simulink model "gtm_design"  (R2021b)
settings: Solver=VariableStepAuto  StartTime=0.0  StopTime=10.0  MinStep=0.00999  RelTol=1e-3
StopFcn:
  | MWSout=grabmws(bdroot);
  | MWSout.lastrun=datestr(now);
values from neighbouring files (symbols this model uses):
  knots2fps = 1.68781    [setup.m]
  s = tf('s')    [setup.m]
undefined symbols (not defined in the file or in its folder): Aero, aftfuel, aftfuel_pos, AILL, AILLC, AILR, AILRC, alpha_deg, alt0, altitude_ft, Ax_g, Ay_g, Az_g, b, beta_deg, bias, BRAKEC, Cbar, cg_pos0, cg_shift_gear, ControlMode, DamageCase, DamageModels, DamageOnsetTime, deltc, Earth, ELLIB, ELLIBC, ELLOB, ELLOBC, ELRIB, ELRIBC, ELROB, ELROBC, engl_ang, engl_pos, engr_ang, engr_pos, etas0, etas1, etasc_feedthrough, FLAPLC, FLAPLIB, FLAPLOB, FLAPRC, FLAPRIB, FLAPROB, FlightMode, FuelUsed_Init, fwdfuel, fwdfuel_pos, GEAR, GEARC, Inertia0, Inertia_shift_gear, Ixx_model, Iyy_model, Izz_model, KTAS, LandingGear ... (+66)
libraries: simulink_extras x98, LPVBlockLibrary x54, simulink_need_slupdate x30, aerolibconvert2 x27, simulink x7, aerolibtransform2 x6, uavalgslib x4, UserContent_lib x2, robotcorelib x1, uavutilslib x1
(part 9 of 9)

== system gtm_design/Control/Controller/Control Algorithm/LPV Autopilot/Longitudinal Controller/Scheduling Parameter ==
  feedback : Inport
  Add : Sum
  Bus Selector1 : BusSelector  OutputSignals=AirData.KTAS,MIDG.NAV_altitude_m,SurfacePos.FLAPLOB,SurfacePos.FLAPROB  OutputAsBus=on
  Bus to Vector : BusToVector
  Demux : Demux
  Gain : Gain  Gain=0.5
  Length Conversion : aerolibconvert2/Length Conversion  IU=m  OU=ft
  MATLAB Function : MATLAB Function  TreatAsAtomicUnit=on
  Mux : Mux  Inputs=3
  rho : Outport
  wires:
  feedback/1 -> Bus Selector1/1
  Bus Selector1/1 -> Bus to Vector/1
  Demux/3 -> Add/1
  Demux/1 -> MATLAB Function/1(tas)
  Demux/4 -> Add/2
  MATLAB Function/1(sas) -> Mux/1  "sas"
  Add/1 -> Gain/1
  Gain/1 -> Mux/3  "mor"
  Demux/2 -> Length Conversion/1  "alt"
  Bus to Vector/1 -> Demux/1
  Mux/1 -> rho/1
  Length Conversion/1 -> MATLAB Function/2(h), Mux/2

== system gtm_design/Control/Controller/Control Algorithm/LPV Autopilot/Longitudinal Controller/Trim Command ==
  rho : Inport
  Constant4 : Constant
  Constant5 : Constant
  LPVBlock1 : LPVBlockLibrary/LPVBlock  sys=sch_param.sch_alt_trim  plist={'rho1_sas_param';'rho2_alt_param';'rho3_mor_param'}  x0=0
      settings: SourceProductName=LPVTools Blocks
  LPVBlock2 : LPVBlockLibrary/LPVBlock  sys=sch_param.sch_tas_trim  plist={'rho1_sas_param';'rho2_alt_param';'rho3_mor_param'}  x0=0
      settings: SourceProductName=LPVTools Blocks
  Mux : Mux  Inputs=2
  knotstofps : Gain  Gain=knots2fps
  r_eq : Outport
  wires:
  Mux/1 -> r_eq/1
  Constant5/1 -> LPVBlock2/1
  LPVBlock2/1 -> knotstofps/1  "tas_trim_knot"
  LPVBlock1/1 -> Mux/2  "alt_trim_ft"
  Constant4/1 -> LPVBlock1/1
  rho/1 -> LPVBlock2/2, LPVBlock1/2
  knotstofps/1 -> Mux/1  "tas_trim_fps"

== system gtm_design/Control/Controller/Control Algorithm/LPV Autopilot/Longitudinal Controller/Trim Input ==
  rho : Inport
  Constant1 : Constant
  Constant3 : Constant
  Mux : Mux  Inputs=2
  dele_trim : LPVBlockLibrary/LPVBlock  sys=sch_param.sch_elevator_trim  plist={'rho1_sas_param';'rho2_alt_param';'rho3_mor_param'}  x0=0
      settings: SourceProductName=LPVTools Blocks
  delt_trim : LPVBlockLibrary/LPVBlock  sys=sch_param.sch_throttle_trim  plist={'rho1_sas_param';'rho2_alt_param';'rho3_mor_param'}  x0=0
      settings: SourceProductName=LPVTools Blocks
  u_eq : Outport
  wires:
  Constant3/1 -> dele_trim/1
  dele_trim/1 -> Mux/2  "dele_trim_deg"
  rho/1 -> dele_trim/2, delt_trim/2
  delt_trim/1 -> Mux/1  "delt_trim_percent"
  Constant1/1 -> delt_trim/1
  Mux/1 -> u_eq/1

== system gtm_design/Control/Controller/Control Algorithm/LPV Autopilot/Longitudinal Controller/Trim State ==
  rho : Inport
  Constant{2..6} (5 alike) : Constant
  Degrees to Radians : simulink_extras/Transformations/Degrees to Radians
  Degrees to Radians1 : simulink_extras/Transformations/Degrees to Radians
  Degrees to Radians2 : simulink_extras/Transformations/Degrees to Radians
  LPVBlock : LPVBlockLibrary/LPVBlock  sys=sch_param.sch_alp_trim  plist={'rho1_sas_param';'rho2_alt_param';'rho3_mor_param'}  x0=0
      settings: SourceProductName=LPVTools Blocks
  LPVBlock1 : LPVBlockLibrary/LPVBlock  sys=sch_param.sch_alt_trim  plist={'rho1_sas_param';'rho2_alt_param';'rho3_mor_param'}  x0=0
      settings: SourceProductName=LPVTools Blocks
  LPVBlock2 : LPVBlockLibrary/LPVBlock  sys=sch_param.sch_tas_trim  plist={'rho1_sas_param';'rho2_alt_param';'rho3_mor_param'}  x0=0
      settings: SourceProductName=LPVTools Blocks
  LPVBlock3 : LPVBlockLibrary/LPVBlock  sys=sch_param.sch_qdeg_trim  plist={'rho1_sas_param';'rho2_alt_param';'rho3_mor_param'}  x0=0
      settings: SourceProductName=LPVTools Blocks
  Mux : Mux  Inputs=5
  knotstofps : Gain  Gain=knots2fps
  sch_pitch_trim : LPVBlockLibrary/LPVBlock  sys=sch_param.sch_pitch_trim  plist={'rho1_sas_param';'rho2_alt_param';'rho3_mor_param'}  x0=0
      settings: SourceProductName=LPVTools Blocks
  x_eq : Outport
  wires:
  Constant5/1 -> LPVBlock2/1
  LPVBlock1/1 -> Mux/5  "alt_trim_deg"
  Constant4/1 -> LPVBlock1/1
  Mux/1 -> x_eq/1
  Degrees to Radians1/1 -> Mux/4  "theta_trim_rad"
  Constant3/1 -> sch_pitch_trim/1
  sch_pitch_trim/1 -> Degrees to Radians1/1  "theta_trim_deg"
  LPVBlock/1 -> Degrees to Radians/1  "alp_trim_deg"
  Constant2/1 -> LPVBlock/1
  LPVBlock2/1 -> knotstofps/1  "tas_trim_knot"
  Degrees to Radians/1 -> Mux/2  "alp_trim_rad"
  knotstofps/1 -> Mux/1  "tas_trim_fps"
  Constant6/1 -> LPVBlock3/1
  rho/1 -> LPVBlock/2, LPVBlock3/2, sch_pitch_trim/2, LPVBlock1/2, LPVBlock2/2
  LPVBlock3/1 -> Degrees to Radians2/1  "q_trim_deg"
  Degrees to Radians2/1 -> Mux/3  "q_trim_rad"

== system gtm_design/Control/Controller/Control Algorithm/LPV CAS/Lateral-Directional Controller/Full State ==
  feedback : Inport
  Bus Selector : BusSelector  OutputSignals=AirData.beta_deg,MAG3.p_deg,MAG3.r_deg
  Degrees to Radians : simulink_extras/Transformations/Degrees to Radians
  Degrees to Radians1 : simulink_extras/Transformations/Degrees to Radians
  Degrees to Radians2 : simulink_extras/Transformations/Degrees to Radians
  Mux : Mux  Inputs=3
  x : Outport
  wires:
  feedback/1 -> Bus Selector/1
  Bus Selector/1 -> Degrees to Radians2/1  "<beta_deg>"
  Bus Selector/2 -> Degrees to Radians/1  "<p_deg>"
  Bus Selector/3 -> Degrees to Radians1/1  "<r_deg>"
  Degrees to Radians1/1 -> Mux/3  "r_rad"
  Degrees to Radians/1 -> Mux/2  "p_rad"
  Degrees to Radians2/1 -> Mux/1  "bet_rad"
  Mux/1 -> x/1

== system gtm_design/Control/Controller/Control Algorithm/LPV CAS/Lateral-Directional Controller/Scheduling Parameter ==
  feedback : Inport
  Add : Sum
  Bus Selector1 : BusSelector  OutputSignals=AirData.KTAS,MIDG.NAV_altitude_m,SurfacePos.FLAPLOB,SurfacePos.FLAPROB  OutputAsBus=on
  Bus to Vector : BusToVector
  Demux : Demux
  Gain : Gain  Gain=0.5
  Length Conversion : aerolibconvert2/Length Conversion  IU=m  OU=ft
  MATLAB Function : MATLAB Function  TreatAsAtomicUnit=on
  Mux : Mux  Inputs=3
  rho : Outport
  wires:
  feedback/1 -> Bus Selector1/1
  Bus Selector1/1 -> Bus to Vector/1
  Demux/3 -> Add/1
  Demux/1 -> MATLAB Function/1(tas)
  Demux/4 -> Add/2
  MATLAB Function/1(sas) -> Mux/1  "sas"
  Add/1 -> Gain/1
  Gain/1 -> Mux/3  "mor"
  Demux/2 -> Length Conversion/1  "alt"
  Bus to Vector/1 -> Demux/1
  Mux/1 -> rho/1
  Length Conversion/1 -> MATLAB Function/2(h), Mux/2

== system gtm_design/Control/Controller/Control Algorithm/LPV CAS/Lateral-Directional Controller/Trim Command ==
  rho : Inport
  Constant : Constant  Value=0
  Constant1 : Constant  Value=0
  Degrees to Radians : simulink_extras/Transformations/Degrees to Radians
  Degrees to Radians1 : simulink_extras/Transformations/Degrees to Radians
  Mux : Mux  Inputs=2
  Terminator : Terminator
  r_eq : Outport
  wires:
  Degrees to Radians1/1 -> Mux/2
  Degrees to Radians/1 -> Mux/1
  Constant1/1 -> Degrees to Radians1/1  "p_trim"
  Constant/1 -> Degrees to Radians/1  "bet_trim"
  rho/1 -> Terminator/1
  Mux/1 -> r_eq/1

== system gtm_design/Control/Controller/Control Algorithm/LPV CAS/Lateral-Directional Controller/Trim Input ==
  rho : Inport
  Constant1 : Constant  Value=0
  Constant2 : Constant
  Constant3 : Constant
  LPVBlock : LPVBlockLibrary/LPVBlock  sys=sch_param.sch_aileron_trim  plist={'rho1_sas_param';'rho2_alt_param';'rho3_mor_param'}  x0=0
      settings: SourceProductName=LPVTools Blocks
  LPVBlock1 : LPVBlockLibrary/LPVBlock  sys=sch_param.sch_rudder_trim  plist={'rho1_sas_param';'rho2_alt_param';'rho3_mor_param'}  x0=0
      settings: SourceProductName=LPVTools Blocks
  Mux : Mux  Inputs=3
  x_eq : Outport
  wires:
  Constant3/1 -> LPVBlock1/1
  Mux/1 -> x_eq/1
  rho/1 -> LPVBlock/2, LPVBlock1/2
  Constant2/1 -> LPVBlock/1
  LPVBlock1/1 -> Mux/2  "delr_trim_deg"
  Constant1/1 -> Mux/3  "etaa_trim_deg"
  LPVBlock/1 -> Mux/1  "dela_trim_deg"

== system gtm_design/Control/Controller/Control Algorithm/LPV CAS/Lateral-Directional Controller/Trim State ==
  rho : Inport
  Constant1 : Constant
  Constant2 : Constant
  Constant3 : Constant
  Degrees to Radians : simulink_extras/Transformations/Degrees to Radians
  Degrees to Radians1 : simulink_extras/Transformations/Degrees to Radians
  Degrees to Radians2 : simulink_extras/Transformations/Degrees to Radians
  LPVBlock : LPVBlockLibrary/LPVBlock  sys=sch_param.sch_beta_trim  plist={'rho1_sas_param';'rho2_alt_param';'rho3_mor_param'}  x0=0
      settings: SourceProductName=LPVTools Blocks
  LPVBlock1 : LPVBlockLibrary/LPVBlock  sys=sch_param.sch_pdeg_trim  plist={'rho1_sas_param';'rho2_alt_param';'rho3_mor_param'}  x0=0
      settings: SourceProductName=LPVTools Blocks
  LPVBlock2 : LPVBlockLibrary/LPVBlock  sys=sch_param.sch_rdeg_trim  plist={'rho1_sas_param';'rho2_alt_param';'rho3_mor_param'}  x0=0
      settings: SourceProductName=LPVTools Blocks
  Mux : Mux  Inputs=3
  x_eq : Outport
  wires:
  Degrees to Radians/1 -> Mux/1  "beta_trim_rad"
  Constant2/1 -> LPVBlock/1
  LPVBlock/1 -> Degrees to Radians/1  "beta_trim_deg"
  LPVBlock1/1 -> Degrees to Radians1/1  "p_trim_deg"
  rho/1 -> LPVBlock2/2, LPVBlock1/2, LPVBlock/2
  Mux/1 -> x_eq/1
  Degrees to Radians1/1 -> Mux/2  "p_trim_rad"
  Constant3/1 -> LPVBlock1/1
  Constant1/1 -> LPVBlock2/1
  LPVBlock2/1 -> Degrees to Radians2/1  "r_trim_deg"
  Degrees to Radians2/1 -> Mux/3  "r_trim_rad"

== system gtm_design/Control/Controller/Control Algorithm/LPV CAS/Longitudinal Controller/Full State ==
  feedback : Inport
  Bus Selector : BusSelector  OutputSignals=AirData.alpha_deg,MAG3.q_deg,MAG3.Az_g
  Degrees to Radians : simulink_extras/Transformations/Degrees to Radians
  Degrees to Radians1 : simulink_extras/Transformations/Degrees to Radians
  Mux : Mux  Inputs=3
  knotstofps : Gain  Gain=32.174
  y : Outport
  wires:
  knotstofps/1 -> Mux/3  "Az_ft/s^2"
  Degrees to Radians1/1 -> Mux/2  "q_rad"
  Degrees to Radians/1 -> Mux/1  "alp_rad"
  Mux/1 -> y/1
  Bus Selector/3 -> knotstofps/1  "<Az_g>"
  Bus Selector/2 -> Degrees to Radians1/1  "<q_deg>"
  Bus Selector/1 -> Degrees to Radians/1  "<alpha_deg>"
  feedback/1 -> Bus Selector/1

== system gtm_design/Control/Controller/Control Algorithm/LPV CAS/Longitudinal Controller/Scheduling Parameter ==
  feedback : Inport
  Add : Sum
  Bus Selector1 : BusSelector  OutputSignals=AirData.KTAS,MIDG.NAV_altitude_m,SurfacePos.FLAPLOB,SurfacePos.FLAPROB  OutputAsBus=on
  Bus to Vector : BusToVector
  Demux : Demux
  Gain : Gain  Gain=0.5
  Length Conversion : aerolibconvert2/Length Conversion  IU=m  OU=ft
  MATLAB Function : MATLAB Function  TreatAsAtomicUnit=on
  Mux : Mux  Inputs=3
  rho : Outport
  wires:
  Length Conversion/1 -> Mux/2, MATLAB Function/2(h)
  Mux/1 -> rho/1
  Bus to Vector/1 -> Demux/1
  Demux/2 -> Length Conversion/1  "alt"
  Gain/1 -> Mux/3  "mor"
  Add/1 -> Gain/1
  MATLAB Function/1(sas) -> Mux/1  "sas"
  Demux/4 -> Add/2
  Demux/1 -> MATLAB Function/1(tas)
  Demux/3 -> Add/1
  Bus Selector1/1 -> Bus to Vector/1
  feedback/1 -> Bus Selector1/1

== system gtm_design/Control/Controller/Control Algorithm/LPV CAS/Longitudinal Controller/Trim Command ==
  rho : Inport
  Constant : Constant
  Terminator : Terminator
  knotstofps : Gain  Gain=32.174
  r_eq : Outport
  wires:
  knotstofps/1 -> r_eq/1  "r"
  Constant/1 -> knotstofps/1
  rho/1 -> Terminator/1

== system gtm_design/Control/Controller/Control Algorithm/LPV CAS/Longitudinal Controller/Trim Input ==
  rho : Inport
  Constant3 : Constant
  dele_trim : LPVBlockLibrary/LPVBlock  sys=sch_param.sch_elevator_trim  plist={'rho1_sas_param';'rho2_alt_param';'rho3_mor_param'}  x0=0
      settings: SourceProductName=LPVTools Blocks
  u_eq : Outport
  wires:
  rho/1 -> dele_trim/2
  dele_trim/1 -> u_eq/1  "dele_trim_deg"
  Constant3/1 -> dele_trim/1

== system gtm_design/Control/Controller/Control Algorithm/LPV CAS/Longitudinal Controller/Trim State ==
  rho : Inport
  Constant : Constant  Value=-1
  Constant2 : Constant
  Constant3 : Constant
  Degrees to Radians : simulink_extras/Transformations/Degrees to Radians
  Degrees to Radians1 : simulink_extras/Transformations/Degrees to Radians
  LPVBlock : LPVBlockLibrary/LPVBlock  sys=sch_param.sch_alp_trim  plist={'rho1_sas_param';'rho2_alt_param';'rho3_mor_param'}  x0=0
      settings: SourceProductName=LPVTools Blocks
  LPVBlock1 : LPVBlockLibrary/LPVBlock  sys=sch_param.sch_qdeg_trim  plist={'rho1_sas_param';'rho2_alt_param';'rho3_mor_param'}  x0=0
      settings: SourceProductName=LPVTools Blocks
  Mux : Mux  Inputs=3
  knotstofps : Gain  Gain=32.174
  x_eq : Outport
  wires:
  Degrees to Radians/1 -> Mux/1  "alp_trim_rad"
  Constant2/1 -> LPVBlock/1
  LPVBlock/1 -> Degrees to Radians/1  "alp_trim_deg"
  LPVBlock1/1 -> Degrees to Radians1/1  "q_trim_deg"
  rho/1 -> LPVBlock1/2, LPVBlock/2
  Mux/1 -> x_eq/1
  Constant/1 -> knotstofps/1  "az_trim_g"
  knotstofps/1 -> Mux/3  "az_trim_ft/s^2"
  Degrees to Radians1/1 -> Mux/2  "q_trim_rad"
  Constant3/1 -> LPVBlock1/1

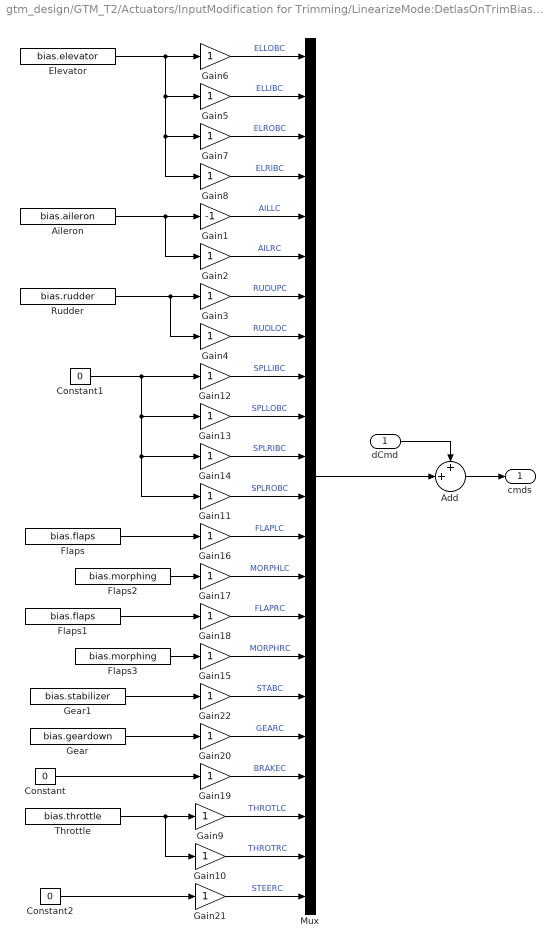
== system gtm_design/GTM_T2/Actuators/InputModification for Trimming/LinearizeMode:DetlasOnTrimBias/Surface Allocation For Linearizing/BiasSurfs ==
  dCmd : Inport
  Add : Sum  Inputs=++|
  Aileron : Constant  Value=bias.aileron
  Constant : Constant  Value=0
  Constant1 : Constant  Value=0
  Constant2 : Constant  Value=0
  Elevator : Constant  Value=bias.elevator
  Flaps : Constant  Value=bias.flaps
  Flaps1 : Constant  Value=bias.flaps
  Flaps2 : Constant  Value=bias.morphing
  Flaps3 : Constant  Value=bias.morphing
  Gain1 : Gain  Gain=-1  SaturateOnIntegerOverflow=on  OutDataTypeStr=Inherit: Same as input  ParamDataTypeStr=Inherit: Same as input
  Gain{2..22} (21 alike) : Gain  SaturateOnIntegerOverflow=on  OutDataTypeStr=Inherit: Same as input  ParamDataTypeStr=Inherit: Same as input
  Gear : Constant  Value=bias.geardown
  Gear1 : Constant  Value=bias.stabilizer
  Mux : Mux  Inputs=22
  Rudder : Constant  Value=bias.rudder
  Throttle : Constant  Value=bias.throttle
  cmds : Outport
  wires:
  Gain21/1 -> Mux/22  "STEERC"
  Constant2/1 -> Gain21/1
  Throttle/1 -> Gain10/1, Gain9/1
  Gain10/1 -> Mux/21  "THROTRC"
  Gain9/1 -> Mux/20  "THROTLC"
  Add/1 -> cmds/1
  dCmd/1 -> Add/1
  Mux/1 -> Add/2
  Gain22/1 -> Mux/17  "STABC"
  Gear1/1 -> Gain22/1
  Aileron/1 -> Gain2/1, Gain1/1
  Gain2/1 -> Mux/6  "AILRC"
  Gain1/1 -> Mux/5  "AILLC"
  Gain20/1 -> Mux/18  "GEARC"
  Constant/1 -> Gain19/1
  Gear/1 -> Gain20/1
  Gain19/1 -> Mux/19  "BRAKEC"
  Flaps/1 -> Gain16/1
  Rudder/1 -> Gain4/1, Gain3/1
  Elevator/1 -> Gain8/1, Gain7/1, Gain5/1, Gain6/1
  Gain4/1 -> Mux/8  "RUDLOC"
  Gain3/1 -> Mux/7  "RUDUPC"
  Gain8/1 -> Mux/4  "ELRIBC"
  Gain7/1 -> Mux/3  "ELROBC"
  Gain6/1 -> Mux/1  "ELLOBC"
  Gain5/1 -> Mux/2  "ELLIBC"
  Gain15/1 -> Mux/16  "MORPHRC"
  Gain18/1 -> Mux/15  "FLAPRC"
  Gain17/1 -> Mux/14  "MORPHLC"
  Gain16/1 -> Mux/13  "FLAPLC"
  Gain11/1 -> Mux/12  "SPLROBC"
  Gain14/1 -> Mux/11  "SPLRIBC"
  Gain13/1 -> Mux/10  "SPLLOBC"
  Gain12/1 -> Mux/9  "SPLLIBC"
  Constant1/1 -> Gain13/1, Gain11/1, Gain14/1, Gain12/1
  Flaps2/1 -> Gain17/1
  Flaps1/1 -> Gain18/1
  Flaps3/1 -> Gain15/1

== system gtm_design/GTM_T2/Actuators/InputModification for Trimming/TrimMode: DriveFromTopLevel/MapPitchSurf/UseElevatorToTrim ==
  In : Inport
  Action Port : ActionPort  ActionPortLabel=default:
  Constant1 : Constant  Value=bias.stabilizer
  Gain : Gain  Gain=[1;1;1;1]
  Mux : Mux  Inputs=[4 1]
  Out : Outport  InitialOutput=[0;0;0;0;bias.stabilizer]
  wires:
  Mux/1 -> Out/1
  Gain/1 -> Mux/1
  Constant1/1 -> Mux/2
  In/1 -> Gain/1

== system gtm_design/GTM_T2/Actuators/InputModification for Trimming/TrimMode: DriveFromTopLevel/MapPitchSurf/UseStabToTrim ==
  In : Inport
  Action Port : ActionPort  ActionPortLabel=case [ 1 ]:
  Constant1 : Constant  Value=bias.elevator
  Gain2 : Gain  Gain=[1;1;1;1]
  Mux : Mux  Inputs=[4 1]
  Out1 : Outport  InitialOutput=[bias.elevator*[1;1;1;1];0]
  wires:
  Mux/1 -> Out1/1
  Gain2/1 -> Mux/1
  In/1 -> Mux/2
  Constant1/1 -> Gain2/1

== matlab function gtm_design/GTM_T2/EOM/Aircraft 6DOF/Form Inertia Matrix ==
  data: Ixx input double size=1; I output size=[3 3]; Iyy input size=1; Izz input size=1; Ixz input size=1; Iyz input size=1; Ixy input size=1; InvI output size=[3 3]
function [I,InvI] = Inertia(Ixx,Iyy,Izz,Ixz,Iyz,Ixy)
% This block supports an embeddable subset of the MATLAB language.
% See the help menu for details. 

I=[ Ixx, -Ixy, -Ixz;
   -Ixy,  Iyy, -Iyz;
   -Ixz, -Iyz,   Izz ];

det = Ixx*Iyy*Izz-Ixx*Iyz^2-Ixy^2*Izz-2*Ixy*Ixz*Iyz-Ixz^2*Iyy;

adjoint=[...
Iyy*Izz-Iyz^2,    Ixy*Izz+Ixz*Iyz, Ixy*Iyz+Ixz*Iyy;...
Ixy*Izz+Ixz*Iyz,   Ixx*Izz-Ixz^2,  Ixx*Iyz+Ixy*Ixz;...
Ixy*Iyz+Ixz*Iyy,  Ixx*Iyz+Ixy*Ixz,   Ixx*Iyy-Ixy^2     ];

InvI=adjoint/det;

== matlab function gtm_design/GTM_T2/Engines/Engine Alignment ==
  data: T output; Tl input; hl input; Tr input; hr input; TL output; engl_ang parameter; engr_ang parameter; TR output; H output
function [T,TL,TR,H] = eng_angles(Tl,hl,Tr,hr,engl_ang,engr_ang)
% This block supports an embeddable subset of the MATLAB language.
% See the help menu for details. 

% Using the engine alignment angles (set in AC_params_T2.m), compute the 
% off-axis thrust and angular momentum terms.

TL = Tl*[cosd(engl_ang(2))*cosd(engl_ang(3));...
         sind(engl_ang(3));...
         -sind(engl_ang(2))*cosd(engl_ang(3))];
TR = Tr*[cosd(engr_ang(2))*cosd(engr_ang(3));...
         sind(engr_ang(3));...
         -sind(engr_ang(2))*cosd(engr_ang(3))];  
T = TL+TR;

H = hl*[cosd(engl_ang(2))*cosd(engl_ang(3));...
         sind(engl_ang(3));...
         -sind(engl_ang(2))*cosd(engl_ang(3))] + ...
         hr*[cosd(engr_ang(2))*cosd(engr_ang(3));...
         sind(engr_ang(3));...
         -sind(engr_ang(2))*cosd(engr_ang(3))];

== matlab function gtm_design/GTM_T2/Engines/Left_Engine Jetcat P70/Simple Ram Drag Model ==
  data: ram_drag output; qbar input; S input; ram_drag_coef parameter
function ram_drag =   ram_drag(qbar,S,ram_drag_coef)
% This block supports the Embedded MATLAB subset.
% See the help menu for details. 

ram_drag = ram_drag_coef.*qbar.*S;
return

== matlab function gtm_design/GTM_T2/Engines/Right_Engine Jetcat P70/Simple Ram Drag Model ==
  data: ram_drag output; qbar input; S input; ram_drag_coef parameter
function ram_drag =   ram_drag(qbar,S,ram_drag_coef)
% This block supports the Embedded MATLAB subset.
% See the help menu for details. 

ram_drag = ram_drag_coef.*qbar.*S;
return

== matlab function gtm_design/Control/Controller/Control Algorithm/Hinf Autopilot/Lateral-Directional Controller/Scheduling Parameter/MATLAB Function ==
  data: tas input; sas output; h input
function sas = fcn(tas, h)
sas = 100-30000/(30000-h)*(100-tas);

== matlab function gtm_design/GTM_T2/A/C parameters/Inertia/Mass/CG Shift/FuelBurnEffects/Polyval1/Embedded MATLAB Function ==
  data: u input; y output; p parameter
function y = fcn(u,p)
% This block supports the Embedded MATLAB subset.
% See the help menu for details. 


y = sum(p.*u.^(length(p)-1:-1:0));

== matlab function gtm_design/Control/Controller/Control Algorithm/Hinf Autopilot/Longitudinal Controller/Scheduling Parameter/MATLAB Function ==
  data: tas input; sas output; h input
function sas = fcn(tas, h)
sas = 100-30000/(30000-h)*(100-tas);

== matlab function gtm_design/Control/Controller/Control Algorithm/Hinf CAS/Lateral-Directional Controller/Scheduling Parameter/MATLAB Function ==
  data: tas input; sas output; h input
function sas = fcn(tas, h)
sas = 100-30000/(30000-h)*(100-tas);

== matlab function gtm_design/Control/Controller/Control Algorithm/LPV Autopilot/Lateral-Directional Controller/Scheduling Parameter/MATLAB Function ==
  data: tas input; sas output; h input
function sas = fcn(tas, h)
sas = 100-30000/(30000-h)*(100-tas);

== matlab function gtm_design/Control/Controller/Control Algorithm/Hinf CAS/Longitudinal Controller/Scheduling Parameter/MATLAB Function ==
  data: tas input; sas output; h input
function sas = fcn(tas, h)
sas = 100-30000/(30000-h)*(100-tas);

== matlab function gtm_design/GTM_T2/A//C parameters/Inertia//Mass//CG Shift/MorphingEffects/MorphingEffectsInertia ==
  data: dinertia output; dCG output; eta input
function [dinertia,dCG]  = fcn(eta)

Cbar    = 0.9153;   % ft,    mean aerodynamic chord
le_mac  = 4.5462;   % ft,    leading edge of MAC
cg_pos0 = [-(le_mac + Cbar*0.2199) -0.1416/12 -0.9761]; % ft, initial CG (21.99% MAC), gear up

lb2slug = 1/32.174;

rcmbar = [cg_pos0(1); cg_pos0(2); cg_pos0(3)]; % [ft]
b = 6.8488; % span [ft]
Lambda = 28.43*pi/180; % sweep [rad]
Gamma = 5*pi/180; % diheral [rad]
m = 57.75*lb2slug; % [slg]
ddm = -0.81*lb2slug; % [slg]
ddrcm = [0.148; 0.628; 0.032]/12; % 3 by 1 [ft]
ddJxx = -0.25821; % slg-ft^2,
ddJyy = -0.01727; % slg-ft^2,
ddJzz = -0.27400; % slg-ft^2,
ddJxz = -0.00295; % slg-ft^2,
ddJyz = -0.01346; % slg-ft^2,
ddJxy = -0.05998; % slg-ft^2,
Jxxbar = 1.221;  % slg-ft^2,
Jyybar = 4.655;  % slg-ft^2,
Jzzbar = 5.587;  % slg-ft^2,
Jxzbar = 0.274;  % slg-ft^2,
Jyzbar = 0.0;    % slg-ft^2,
Jxybar = 0.006;  % slg-ft^2,
ddJ=[ ddJxx, -ddJxy, -ddJxz;
     -ddJxy,  ddJyy, -ddJyz;
     -ddJxz, -ddJyz,  ddJzz ];
Jbar=[Jxxbar, -Jxybar, -Jxzbar;
     -Jxybar,  Jyybar, -Jyzbar;
     -Jxzbar, -Jyzbar,  Jzzbar ];

etal = eta(1); % left morphing [%]
etar = eta(2); % right morphing [%]

ml = -ddm;
mr = ml;
mb = m-ml-mr;

drl = -(etal/25)*[b*tan(Gamma)/8;  b/8; b*tan(Gamma)/(8*cos(Lambda))]; % 3 by 1 
drr = -(etar/25)*[b*tan(Gamma)/8; -b/8; b*tan(Gamma)/(8*cos(Lambda))]; % 3 by 1
drcm = (ml/m)*drl+(mr/m)*drr;
dCG = drcm;
rcm = rcmbar+drcm;

rlbar = rcmbar-(m/ml-1)*ddrcm;
rrbar = diag([1,-1,1])*rlbar;
rbbar = (m*rcmbar-ml*rlbar-mr*rrbar)/mb;

rl = rlbar+drl;
rb = rbbar;
rr = rrbar+drr;

temp1 = rlbar-rcmbar;
temp2 = rbbar-rcmbar;
temp3 = rrbar-rcmbar;
temp4 = rbbar-(rcmbar+ddrcm);
temp5 = rrbar-(rcmbar+ddrcm);

Jlbar = -ddJ...
    -ml*(trace(temp1*temp1.')*eye(3)-temp1*temp1.')...
    -mb*(trace(temp2*temp2.')*eye(3)-temp2*temp2.')...
    -mr*(trace(temp3*temp3.')*eye(3)-temp3*temp3.')...
    +mb*(trace(temp4*temp4.')*eye(3)-temp4*temp4.')...
    +mr*(trace(temp5*temp5.')*eye(3)-temp5*temp5.');
Jlbar=-Jlbar;
Jrbar = [ Jlbar(1,1) -Jlbar(1,2)  Jlbar(1,3);
         -Jlbar(2,1)  Jlbar(2,2) -Jlbar(2,3);
          Jlbar(3,1) -Jlbar(3,2)  Jlbar(3,3)];
temp6 = rlbar-rcmbar;
temp7 = rrbar-rcmbar;
Jbbar = Jbar-Jlbar-ml*(trace((temp6)*(temp6).')*eye(3)-(temp6)*(temp6).')...
            -Jrbar-mr*(trace((temp7)*(temp7).')*eye(3)-(temp7)*(temp7).');
temp8 = rl-rcm;
temp9 = rb-rcm;
temp0 = rr-rcm;
Jl = Jlbar+ml*(trace((temp8)*(temp8).')*eye(3)-(temp8)*(temp8).');
Jb = Jbbar+mb*(trace((temp9)*(temp9).')*eye(3)-(temp9)*(temp9).');
Jr = Jrbar+mr*(trace((temp0)*(temp0).')*eye(3)-(temp0)*(temp0).');
J = Jl+Jb+Jr;
dJ = J-Jbar;
dinertia = [dJ(1,1) dJ(2,2) dJ(3,3) -dJ(1,3) -dJ(2,3) -dJ(1,2)];

== matlab function gtm_design/Guidance/Label/MATLAB Function ==
  data: tas_c_knot input; detas output
function detas = fcn(tas_c_knot)

ind = (tas_c_knot-60)/60;
detas = -25*ind/2;

== matlab function gtm_design/Control/Controller/Control Algorithm/LPV Autopilot/Longitudinal Controller/Scheduling Parameter/MATLAB Function ==
  data: tas input; sas output; h input
function sas = fcn(tas, h)
sas = 100-30000/(30000-h)*(100-tas);

== matlab function gtm_design/Guidance/Orbit Following/Heading Control ==
  data: FlightState input Bus: FixedWingStateBus; UHeading input; RollAngle output size=[1 1]; e input Bus: FixedWingEnvironmentBus
function RollAngle = fcn(FlightState, UHeading, e)

PHeadingAngle = 0.39;

Va = FlightState.AirSpeed;
HeadingAngle = FlightState.HeadingAngle;
FlightPathAngle = FlightState.FlightPathAngle;

YawAngle = HeadingAngle - asin((1/Va)*[e.WindNorth, e.WindEast]*[-sin(HeadingAngle); cos(HeadingAngle)]);
b = [cos(HeadingAngle)*cos(FlightPathAngle), sin(HeadingAngle)*cos(FlightPathAngle), -sin(FlightPathAngle)]*[e.WindNorth; e.WindEast; e.WindDown];
c = [e.WindNorth, e.WindEast, e.WindDown]*[e.WindNorth; e.WindEast; e.WindDown]- Va^2;
Vg = -b+sqrt(b^2-c);

RollAngle = atan2(PHeadingAngle*angdiff(HeadingAngle,UHeading)*Vg,e.Gravity*cos(HeadingAngle-YawAngle));

== matlab function gtm_design/Guidance/Waypoint Following/Heading Control ==
  data: FlightState input Bus: FixedWingStateBus; UHeading input; RollAngle output size=[1 1]; e input Bus: FixedWingEnvironmentBus
function RollAngle = fcn(FlightState, UHeading, e)

PHeadingAngle = 0.39;

Va = FlightState.AirSpeed;
HeadingAngle = FlightState.HeadingAngle;
FlightPathAngle = FlightState.FlightPathAngle;

YawAngle = HeadingAngle - asin((1/Va)*[e.WindNorth, e.WindEast]*[-sin(HeadingAngle); cos(HeadingAngle)]);
b = [cos(HeadingAngle)*cos(FlightPathAngle), sin(HeadingAngle)*cos(FlightPathAngle), -sin(FlightPathAngle)]*[e.WindNorth; e.WindEast; e.WindDown];
c = [e.WindNorth, e.WindEast, e.WindDown]*[e.WindNorth; e.WindEast; e.WindDown]- Va^2;
Vg = -b+sqrt(b^2-c);

RollAngle = atan2(PHeadingAngle*angdiff(HeadingAngle,UHeading)*Vg,e.Gravity*cos(HeadingAngle-YawAngle));

== matlab function gtm_design/Guidance/Heading Control/Heading Control ==
  data: FlightState input Bus: FixedWingStateBus; UHeading input; RollAngle output size=[1 1]; e input Bus: FixedWingEnvironmentBus
function RollAngle = fcn(FlightState, UHeading, e)

PHeadingAngle = 0.39;

Va = FlightState.AirSpeed;
HeadingAngle = FlightState.HeadingAngle;
FlightPathAngle = FlightState.FlightPathAngle;

YawAngle = HeadingAngle - asin((1/Va)*[e.WindNorth, e.WindEast]*[-sin(HeadingAngle); cos(HeadingAngle)]);
b = [cos(HeadingAngle)*cos(FlightPathAngle), sin(HeadingAngle)*cos(FlightPathAngle), -sin(FlightPathAngle)]*[e.WindNorth; e.WindEast; e.WindDown];
c = [e.WindNorth, e.WindEast, e.WindDown]*[e.WindNorth; e.WindEast; e.WindDown]- Va^2;
Vg = -b+sqrt(b^2-c);

RollAngle = atan2(PHeadingAngle*angdiff(HeadingAngle,UHeading)*Vg,e.Gravity*cos(HeadingAngle-YawAngle));

== matlab function gtm_design/GTM_T2/A/C parameters/Inertia/Mass/CG Shift/fuel cg shift, cg_pos0 ==
  data: fuel_used input; y output; aftfuel parameter; fwdfuel parameter; aftfuel_pos parameter; fwdfuel_pos parameter; w0 parameter; cg_pos0 parameter
function y = fcn(fuel_used,aftfuel,fwdfuel,aftfuel_pos,fwdfuel_pos,w0,cg_pos0)
% This block supports an embeddable subset of the MATLAB language.
% See the help menu for details. 

y = w0.*cg_pos0 - min(aftfuel,fuel_used).*aftfuel_pos - max(0,fuel_used-fwdfuel).*fwdfuel_pos;

== matlab function gtm_design/Control/Controller/Control Algorithm/LPV CAS/Lateral-Directional Controller/Scheduling Parameter/MATLAB Function ==
  data: tas input; sas output; h input
function sas = fcn(tas, h)
sas = 100-30000/(30000-h)*(100-tas);

== matlab function gtm_design/Control/Controller/Control Algorithm/LPV CAS/Longitudinal Controller/Scheduling Parameter/MATLAB Function ==
  data: tas input; sas output; h input
function sas = fcn(tas, h)
sas = 100-30000/(30000-h)*(100-tas);

== matlab function gtm_design/Guidance/Label/MATLAB Function1 ==
  data: alt_c_ft input; detas output
function detas = fcn(alt_c_ft)

detas = -25*(10000-alt_c_ft)/10000/2;

== matlab function gtm_design/GTM_T2/A/C parameters/Inertia/Mass/CG Shift/FuelBurnEffects/Polyval2/Embedded MATLAB Function ==
  data: u input; y output; p parameter
function y = fcn(u,p)
% This block supports the Embedded MATLAB subset.
% See the help menu for details. 


y = sum(p.*u.^(length(p)-1:-1:0));

== matlab function gtm_design/GTM_T2/Aero/Control Surfaces/Implement Damage Models/Implement Damage Models ==
  data: SurfVec input; DamageCase input; dC6 output; SurfGain parameter
function dC6 = fcn(SurfVec,DamageCase,SurfGain)
% This block supports an embeddable subset of the MATLAB language.
% See the help menu for details. 
damagecase = cast(round(DamageCase),'uint32');
Nsurfs=18;
if (damagecase==0),
    dC6=ones(1,Nsurfs)*(reshape(SurfVec,6,Nsurfs)');
else
  gain=squeeze(SurfGain(damagecase,:,:));
  dC6=ones(1,Nsurfs)*( transpose(reshape(SurfVec,6,Nsurfs)).*gain);
end

== matlab function gtm_design/GTM_T2/Aero/Dynamic Derviatives/Rotary Blended UnDamaged Case/Blending Function ==
  data: alpha input; omega output; beta input; tas input; pqr input; pqr_osc output; B input; Cbar input
function[omega,pqr_osc]= hykal(alpha,beta,tas,pqr,B,Cbar)
% Hybrid Kalviste blending method for use in embedded block in Simulink.
%
% Austin Murch
% Austin.M.Murch@nasa.gov

% Dimension vector outputs.
pqr_osc=zeros(3,1);
 

% Constants
dtr=pi/180;
knots2ft=1.689;

% Setup variables
pb=pqr(1);
qb=pqr(2);
rb=pqr(3);

alpha = alpha*dtr;
beta = beta*dtr;
omega = 0;

%----Hybrid Kalviste Method----%
whichcase = 0;

%Test for case 1: p_osc = 0
if cos(alpha)*cos(beta) == 0
elseif pb == 0
else
    omega = pb/(cos(alpha)*cos(beta));
    r_osc = rb - omega*sin(alpha)*cos(beta);
    if abs(r_osc) > abs(rb)
    elseif r_osc*rb < 0
    else
        whichcase = 1;
    end
end

%Test for case 2: r_osc = 0
if sin(alpha)*cos(beta) == 0
elseif rb == 0
else
    omega = rb/(sin(alpha)*cos(beta));
    p_osc = pb - omega*cos(alpha)*cos(beta);
    if abs(p_osc) > abs(pb)
    elseif p_osc*pb < 0
    else
        whichcase = 2;
    end
end

%Test for case 3: Omega = 0
if whichcase == 0
    whichcase = 3;
end

 

switch whichcase
    case 1
        omega = pb/(cos(alpha)*cos(beta));
        pqr_osc(1) = 0;        
        pqr_osc(2) = qb - omega*sin(beta);        
        pqr_osc(3) = rb - omega*sin(alpha)*cos(beta);

    case 2
        omega = rb/(sin(alpha)*cos(beta));
        pqr_osc(1) = pb - omega*cos(alpha)*cos(beta);
        pqr_osc(2) = qb - omega*sin(beta);
        pqr_osc(3) = 0;

    case 3
        pqr_osc(1) = pb;
        pqr_osc(2) = qb;
        pqr_osc(3) = rb;
        omega = 0;
end

%-----------------------------------------------% End Hybrid Kalviste

% Scale values for table lookup
b2vt=B/(2*tas*knots2ft);
c2vt=Cbar/(2*tas*knots2ft);
omega=omega*b2vt;
pqr_osc=pqr_osc.*[b2vt;c2vt;b2vt];

== matlab function gtm_design/GTM_T2/A/C parameters/Inertia/Mass/CG Shift/FuelBurnEffects/Polyval/Embedded MATLAB Function ==
  data: u input; y output; p parameter
function y = fcn(u,p)
% This block supports the Embedded MATLAB subset.
% See the help menu for details. 


y = sum(p.*u.^(length(p)-1:-1:0));

== matlab function gtm_design/GTM_T2/AuxiliaryVariables/Atmos76/atmos76 ==
  data: z input; y output; dt input
function y = layer1atm(z,dt)
% Author: Kevin Cunningham          April 20, 1992    
% Modified: Dave Cox                Aug, 14, 2008

y=zeros(6,1);

%dt=0;  % Standard Temp forced.

%    --- constants from 1976 std. atmosphere
r     = 1716.55915670803;
gamma = 1.4;
g     = 32.17405;
re    = 20855531.5;
tsl   = 288.15 * 1.8;
psl   = 2116.22;
hsl   = 0.;
sldens = 0.0023769;                 % atmospheric density at sea level
slpr   = 2116.220;                  % sea level pressure, psf

%---------------------------------------------------------------------
%    conversion from metric lapse rate to english lapse rate
%    meters/0.3048 = ft
%    Kelvin * 1.8 = Rankine
rm2ft = 1000.0/0.3048;
conlapse = 1.8/rm2ft;

%  ---- convert geometric alt. to geopotential alt.
h     = (re*z)/(re+z);
 
%  ---- ensure we are in layer one (based on geopotential alt)
if (h > 11*rm2ft) % 11 km
  %fprintf(1,'Error, atmosphere model out of range %f, Limiting...\n',h);
  h=11*rm2ft;
end
if (h<0)
  %fprintf(1,'Error, atmosphere model out of range %f, Limiting...\n',h);
  h=0;
end

a1     = -6.5*conlapse;
t1     = tsl + a1*(h-hsl);
del1   = (t1/tsl)^(-g/r/a1);
p1     = del1 * psl;

%   ---- apply temperature increment from standard day*/
t1     = t1 + dt;

%   ---- calculate density from eqn. of state w/ corrected temp.*/
rho1   = p1 / (r * t1);
 
%   ---- calculate speed of sound w/ corrected temp.*/
c1     = sqrt(gamma * (r * t1));
 

% Calculate outputs
y(1) = rho1;
y(2) = p1;
y(3) = t1 / 1.8; % output temperature  in Kelvin
y(4) = c1;
y(5) = y(2) / slpr;         % pressure ratio
y(6) = sqrt(y(1)/sldens);   % SQUARE ROOT OF DENSITY RATIO

== matlab function gtm_design/GTM_T2/AuxiliaryVariables/Embedded MATLAB Function ==
  data: omega input; euler input; v input; n_body output; v_dot input
function n_body = accels(omega,euler,v,v_dot)
% Compute body-axis accelerometer measurements.  
% Inputs:
%       omega: body-axis angular rates, [p q r], in rad/sec
%       euler: Euler angles, [phi theta psi], in rad
%           v: body-axis velocities, [u v w], ft/sec
%       v_dot: body-axis accelerations, [udot vdot wdot], ft/sec^2
%
%
% Author: Austin Murch (Austin.M.Murch@nasa.gov)
% Created: 2/19/2008

g0    = 32.174;
phi   = euler(1);
theta = euler(2);

n_body = (v_dot + cross(omega,v))/g0 - [-sin(theta); cos(theta)*sin(phi); cos(theta)*cos(phi)];

== matlab function gtm_design/GTM_T2/EOM/Aircraft 6DOF/EulerDot ==
  data: pqr input size=3; deuler output size=3; euler input size=3
function deuler = e2de(pqr,euler)
% This block supports an embeddable subset of the MATLAB language.
% See the help menu for details. 

P=pqr(1);
Q=pqr(2);
R=pqr(3);

phi=euler(1);
theta=euler(2);
psi=euler(3);

c_phi=cos(phi);
s_phi=sin(phi);
c_theta=cos(theta);
s_theta=sin(theta);

phi_dot   = P + (1/c_theta)*(s_phi*s_theta*Q + c_phi*s_theta*R);
theta_dot = c_phi*Q - s_phi*R;
psi_dot   = (1/c_theta)*(s_phi*Q + c_phi*R);

deuler=[phi_dot; theta_dot; psi_dot];
